simulink model "Main_SpeedOptimisedVersionTannenweg"  (R2024b)
settings: Solver=ode15s  StartTime=0.0  StopTime=3600*2  FixedStep=0.1  RelTol=0.001
model workspace (MAT data in the model file):
  Ti = 5
  fa = 0.00071
  fd = 0.03
  ips = 36
  ma = 0.0013
  md = 0.04
  roomarea1 = 20
  s = 15
libraries: fl_lib x1434, nesl_utility x105, SimscapeFluids_lib x35
(part 19 of 22)

== system Main_SpeedOptimisedVersionTannenweg/OG1/Raum3/X-Atm ==
  Air-Wall Convection : fl_lib/Thermal/Thermal Elements/Convective Heat Transfer  thermal_type=foundation.enum.constant_variable.constant  area=8.7 m^2  heat_tr_coeff=.8 W/m^2/K  min_heat_tr_coeff=1e-3 W/(K*m^2)  T_specify=off  T_priority=High  T=0 K  T_nominal_specify=off  T_nominal_value=1  T_nominal_unit=K  Q_specify=off  Q_priority=High  Q=0 J/s  Q_nominal_specify=off  Q_nominal_value=1  Q_nominal_unit=W
  Air-Window Convection : fl_lib/Thermal/Thermal Elements/Convective Heat Transfer  thermal_type=foundation.enum.constant_variable.constant  area=3 m^2  heat_tr_coeff=.8 W/m^2/K  min_heat_tr_coeff=1e-3 W/(K*m^2)  T_specify=off  T_priority=High  T=0 K  T_nominal_specify=off  T_nominal_value=1  T_nominal_unit=K  Q_specify=off  Q_priority=High  Q=0 J/s  Q_nominal_specify=off  Q_nominal_value=1  Q_nominal_unit=W
  Atm-Wall Convection : fl_lib/Thermal/Thermal Elements/Convective Heat Transfer  thermal_type=foundation.enum.constant_variable.constant  area=8.7 m^2  heat_tr_coeff=25 W/m^2/K  min_heat_tr_coeff=1e-3 W/(K*m^2)  T_specify=off  T_priority=High  T=0 K  T_nominal_specify=off  T_nominal_value=1  T_nominal_unit=K  Q_specify=off  Q_priority=High  Q=0 J/s  Q_nominal_specify=off  Q_nominal_value=1  Q_nominal_unit=W
  Atm-Window Convection : fl_lib/Thermal/Thermal Elements/Convective Heat Transfer  thermal_type=foundation.enum.constant_variable.constant  area=3 m^2  heat_tr_coeff=25 W/m^2/K  min_heat_tr_coeff=1e-3 W/(K*m^2)  T_specify=off  T_priority=High  T=0 K  T_nominal_specify=off  T_nominal_value=1  T_nominal_unit=K  Q_specify=off  Q_priority=High  Q=0 J/s  Q_nominal_specify=off  Q_nominal_value=1  Q_nominal_unit=W
  Half Wall-Air Conduction : fl_lib/Thermal/Thermal Elements/Conductive Heat Transfer  thermal_type=foundation.enum.ConstantVariableTabulated.Constant  wall_geometry=foundation.enum.ConductionWallGeometry.Planar  area=8.7 m^2  thickness=.16 m  d_in=0.05 m  d_out=0.1 m  L=1 m  th_cond_min=10 W/(K*m)  th_cond=.069 W/m/K  th_cond_TLU=[413, 401, 392, 383, 371, 357, 342] W/(K*m)  temp_TLU=[200, 273, 400, 600, 800, 1000, 1200] K  T_specify=off  T_priority=High  T=0 K  T_nominal_specify=off  T_nominal_value=1  T_nominal_unit=K  Q_specify=off  Q_priority=High  Q=0 J/s  Q_nominal_specify=off  Q_nominal_value=1  Q_nominal_unit=W
  Half Wall-Atm Conduction : fl_lib/Thermal/Thermal Elements/Conductive Heat Transfer  thermal_type=foundation.enum.ConstantVariableTabulated.Constant  wall_geometry=foundation.enum.ConductionWallGeometry.Planar  area=8.7 m^2  thickness=.16 m  d_in=0.05 m  d_out=0.1 m  L=1 m  th_cond_min=10 W/(K*m)  th_cond=.069 W/m/K  th_cond_TLU=[413, 401, 392, 383, 371, 357, 342] W/(K*m)  temp_TLU=[200, 273, 400, 600, 800, 1000, 1200] K  T_specify=off  T_priority=High  T=0 K  T_nominal_specify=off  T_nominal_value=1  T_nominal_unit=K  Q_specify=off  Q_priority=High  Q=0 J/s  Q_nominal_specify=off  Q_nominal_value=1  Q_nominal_unit=W
  Half Window-Air Conduction : fl_lib/Thermal/Thermal Elements/Conductive Heat Transfer  thermal_type=foundation.enum.ConstantVariableTabulated.Constant  wall_geometry=foundation.enum.ConductionWallGeometry.Planar  area=3 m^2  thickness=.027 m  d_in=0.05 m  d_out=0.1 m  L=1 m  th_cond_min=10 W/(K*m)  th_cond=.43 W/m/K  th_cond_TLU=[413, 401, 392, 383, 371, 357, 342] W/(K*m)  temp_TLU=[200, 273, 400, 600, 800, 1000, 1200] K  T_specify=off  T_priority=High  T=0 K  T_nominal_specify=off  T_nominal_value=1  T_nominal_unit=K  Q_specify=off  Q_priority=High  Q=0 J/s  Q_nominal_specify=off  Q_nominal_value=1  Q_nominal_unit=W
  Half Window-Atm Conduction : fl_lib/Thermal/Thermal Elements/Conductive Heat Transfer  thermal_type=foundation.enum.ConstantVariableTabulated.Constant  wall_geometry=foundation.enum.ConductionWallGeometry.Planar  area=3 m^2  thickness=.027 m  d_in=0.05 m  d_out=0.1 m  L=1 m  th_cond_min=10 W/(K*m)  th_cond=.43 W/m/K  th_cond_TLU=[413, 401, 392, 383, 371, 357, 342] W/(K*m)  temp_TLU=[200, 273, 400, 600, 800, 1000, 1200] K  T_specify=off  T_priority=High  T=0 K  T_nominal_specify=off  T_nominal_value=1  T_nominal_unit=K  Q_specify=off  Q_priority=High  Q=0 J/s  Q_nominal_specify=off  Q_nominal_value=1  Q_nominal_unit=W
  Thermal Mass Wall : fl_lib/Thermal/Thermal Elements/Thermal Mass  mass_type=foundation.enum.constant_variable.constant  mass=1500 kg  sp_heat=876 J/kg/K  mass_min=1e-6 kg  num_ports=foundation.enum.numPorts2.one  m_specify=off  m_priority=High  m=1 kg  m_nominal_specify=off  m_nominal_value=1  m_nominal_unit=kg  T_specify=on  T_priority=High  T=Ti degC  T_nominal_specify=off  T_nominal_value=1  T_nominal_unit=K  Q_specify=off  Q_priority=None  Q=0 W  Q_nominal_specify=off  Q_nominal_value=1  Q_nominal_unit=W
  Thermal Mass Window : fl_lib/Thermal/Thermal Elements/Thermal Mass  mass_type=foundation.enum.constant_variable.constant  mass=176 kg  sp_heat=884 J/kg/K  mass_min=1e-6 kg  num_ports=foundation.enum.numPorts2.one  m_specify=off  m_priority=High  m=1 kg  m_nominal_specify=off  m_nominal_value=1  m_nominal_unit=kg  T_specify=on  T_priority=High  T=Ti degC  T_nominal_specify=off  T_nominal_value=1  T_nominal_unit=K  Q_specify=off  Q_priority=None  Q=0 W  Q_nominal_specify=off  Q_nominal_value=1  Q_nominal_unit=W
  Conn1 : PMIOPort  Side=Left
  Conn2 : PMIOPort  Port=2  Side=Right
  connections:
  Air-Wall Convection/RConn1 -- Half Wall-Air Conduction/LConn1
  Air-Window Convection/RConn1 -- Half Window-Air Conduction/LConn1
  Half Wall-Atm Conduction/RConn1 -- Atm-Wall Convection/LConn1
  Half Window-Atm Conduction/RConn1 -- Atm-Window Convection/LConn1
  Atm-Wall Convection/RConn1 -- Conn2/RConn1 -- Atm-Window Convection/RConn1
  Half Wall-Atm Conduction/LConn1 -- Half Wall-Air Conduction/RConn1 -- Thermal Mass Wall/LConn1
  Half Window-Atm Conduction/LConn1 -- Half Window-Air Conduction/RConn1 -- Thermal Mass Window/LConn1
  Conn1/RConn1 -- Air-Wall Convection/LConn1 -- Air-Window Convection/LConn1

== system Main_SpeedOptimisedVersionTannenweg/OG1/Raum4/Heater ==
  valve command : Inport
  Gate Valve (TL)1 : SimscapeFluids_lib/Thermal Liquid/Valves & Orifices/Flow Control Valves/Gate Valve (TL)  diam_orifice=fd m  S_min=0 m  area_leak=1e-10 m^2  smoothing_factor=0.01  area=fa m^2  Cd=0.64  Re_c=150
      settings: InternalSimscapePortConfiguration="{\"Bottom\":[],\"Left\":[{\"id\":\"A\",\"label\":\"A\",\"type\":\"foundation.thermal_liquid.thermal_liquid\"},{\"id\":\"S\",\"label\":\"S\",\"type\":\"input\"}],\"Right\":[{\"id\":\"B\",\"label\":\"B\",\"type\":\"foundation.thermal_liquid.thermal_liquid\"}],\"Top\":[]}"
  Subsystem : Subsystem
  heating panel typ 11 : fl_lib/Thermal Liquid/Elements/Pipe (TL)  length=5 m  area=0.01 m^2  Dh=0.1128 m  length_add=1 m  roughness=15e-6 m  Re_lam=2000  Re_tur=4000  shape_factor=64  Nu_lam=3.66  dynamic_compressibility=true  inertia=false  p0=0.101325 MPa  T0=293.15 K  mdot0=0 kg/s
  Water in : PMIOPort  Side=Left
  Heat : PMIOPort  Port=2  Side=Right
  water out : PMIOPort  Port=3  Side=Right
  wires:
  valve command/1 -> Subsystem/1(VCmd)
  connections:
  heating panel typ 11/RConn1 -- water out/RConn1
  Gate Valve (TL)1/RConn1 -- heating panel typ 11/LConn1
  heating panel typ 11/LConn2 -- Heat/RConn1
  Gate Valve (TL)1/LConn2 -- Subsystem/RConn1
  Water in/RConn1 -- Gate Valve (TL)1/LConn1

== system Main_SpeedOptimisedVersionTannenweg/OG1/Raum4/Temp. Sensor ==
  PS2S : nesl_utility/PS-Simulink Converter  PhysicalDomain=network_engine_domain  SubClassName=ps_output  LeftPortType=input  RightPortType=output  PseudoPeriodic=off  Frequencies=[]  VectorFormat=1-D array  Unit=degC  AffineConversion=on
  TRef : fl_lib/Thermal/Thermal Elements/Thermal Reference
  Temperature Sensor : fl_lib/Thermal/Thermal Sensors/Temperature Sensor  temperature_measure=foundation.enum.MeasurementReference.difference
  Pr : PMIOPort  Side=Left
  T : Outport  VectorParamsAs1DForOutWhenUnconnected=off
  wires:
  PS2S/1 -> T/1
  connections:
  Temperature Sensor/RConn1 -- TRef/LConn1
  PS2S/LConn1 -- Temperature Sensor/RConn2
  Pr/RConn1 -- Temperature Sensor/LConn1

== system Main_SpeedOptimisedVersionTannenweg/OG1/Raum4/X-Atm ==
  Air-Wall Convection : fl_lib/Thermal/Thermal Elements/Convective Heat Transfer  thermal_type=foundation.enum.constant_variable.constant  area=4 m^2  heat_tr_coeff=.8 W/m^2/K  min_heat_tr_coeff=1e-3 W/(K*m^2)  T_specify=off  T_priority=High  T=0 K  T_nominal_specify=off  T_nominal_value=1  T_nominal_unit=K  Q_specify=off  Q_priority=High  Q=0 J/s  Q_nominal_specify=off  Q_nominal_value=1  Q_nominal_unit=W
  Air-Window Convection : fl_lib/Thermal/Thermal Elements/Convective Heat Transfer  thermal_type=foundation.enum.constant_variable.constant  area=1.3 m^2  heat_tr_coeff=.8 W/m^2/K  min_heat_tr_coeff=1e-3 W/(K*m^2)  T_specify=off  T_priority=High  T=0 K  T_nominal_specify=off  T_nominal_value=1  T_nominal_unit=K  Q_specify=off  Q_priority=High  Q=0 J/s  Q_nominal_specify=off  Q_nominal_value=1  Q_nominal_unit=W
  Atm-Wall Convection : fl_lib/Thermal/Thermal Elements/Convective Heat Transfer  thermal_type=foundation.enum.constant_variable.constant  area=4 m^2  heat_tr_coeff=25 W/m^2/K  min_heat_tr_coeff=1e-3 W/(K*m^2)  T_specify=off  T_priority=High  T=0 K  T_nominal_specify=off  T_nominal_value=1  T_nominal_unit=K  Q_specify=off  Q_priority=High  Q=0 J/s  Q_nominal_specify=off  Q_nominal_value=1  Q_nominal_unit=W
  Atm-Window Convection : fl_lib/Thermal/Thermal Elements/Convective Heat Transfer  thermal_type=foundation.enum.constant_variable.constant  area=1.3 m^2  heat_tr_coeff=25 W/m^2/K  min_heat_tr_coeff=1e-3 W/(K*m^2)  T_specify=off  T_priority=High  T=0 K  T_nominal_specify=off  T_nominal_value=1  T_nominal_unit=K  Q_specify=off  Q_priority=High  Q=0 J/s  Q_nominal_specify=off  Q_nominal_value=1  Q_nominal_unit=W
  Half Wall-Air Conduction : fl_lib/Thermal/Thermal Elements/Conductive Heat Transfer  thermal_type=foundation.enum.ConstantVariableTabulated.Constant  wall_geometry=foundation.enum.ConductionWallGeometry.Planar  area=4 m^2  thickness=.16 m  d_in=0.05 m  d_out=0.1 m  L=1 m  th_cond_min=10 W/(K*m)  th_cond=.069 W/m/K  th_cond_TLU=[413, 401, 392, 383, 371, 357, 342] W/(K*m)  temp_TLU=[200, 273, 400, 600, 800, 1000, 1200] K  T_specify=off  T_priority=High  T=0 K  T_nominal_specify=off  T_nominal_value=1  T_nominal_unit=K  Q_specify=off  Q_priority=High  Q=0 J/s  Q_nominal_specify=off  Q_nominal_value=1  Q_nominal_unit=W
  Half Wall-Atm Conduction : fl_lib/Thermal/Thermal Elements/Conductive Heat Transfer  thermal_type=foundation.enum.ConstantVariableTabulated.Constant  wall_geometry=foundation.enum.ConductionWallGeometry.Planar  area=4 m^2  thickness=.16 m  d_in=0.05 m  d_out=0.1 m  L=1 m  th_cond_min=10 W/(K*m)  th_cond=.069 W/m/K  th_cond_TLU=[413, 401, 392, 383, 371, 357, 342] W/(K*m)  temp_TLU=[200, 273, 400, 600, 800, 1000, 1200] K  T_specify=off  T_priority=High  T=0 K  T_nominal_specify=off  T_nominal_value=1  T_nominal_unit=K  Q_specify=off  Q_priority=High  Q=0 J/s  Q_nominal_specify=off  Q_nominal_value=1  Q_nominal_unit=W
  Half Window-Air Conduction : fl_lib/Thermal/Thermal Elements/Conductive Heat Transfer  thermal_type=foundation.enum.ConstantVariableTabulated.Constant  wall_geometry=foundation.enum.ConductionWallGeometry.Planar  area=1.3 m^2  thickness=.027 m  d_in=0.05 m  d_out=0.1 m  L=1 m  th_cond_min=10 W/(K*m)  th_cond=.43 W/m/K  th_cond_TLU=[413, 401, 392, 383, 371, 357, 342] W/(K*m)  temp_TLU=[200, 273, 400, 600, 800, 1000, 1200] K  T_specify=off  T_priority=High  T=0 K  T_nominal_specify=off  T_nominal_value=1  T_nominal_unit=K  Q_specify=off  Q_priority=High  Q=0 J/s  Q_nominal_specify=off  Q_nominal_value=1  Q_nominal_unit=W
  Half Window-Atm Conduction : fl_lib/Thermal/Thermal Elements/Conductive Heat Transfer  thermal_type=foundation.enum.ConstantVariableTabulated.Constant  wall_geometry=foundation.enum.ConductionWallGeometry.Planar  area=1.3 m^2  thickness=.027 m  d_in=0.05 m  d_out=0.1 m  L=1 m  th_cond_min=10 W/(K*m)  th_cond=.43 W/m/K  th_cond_TLU=[413, 401, 392, 383, 371, 357, 342] W/(K*m)  temp_TLU=[200, 273, 400, 600, 800, 1000, 1200] K  T_specify=off  T_priority=High  T=0 K  T_nominal_specify=off  T_nominal_value=1  T_nominal_unit=K  Q_specify=off  Q_priority=High  Q=0 J/s  Q_nominal_specify=off  Q_nominal_value=1  Q_nominal_unit=W
  Thermal Mass Wall : fl_lib/Thermal/Thermal Elements/Thermal Mass  mass_type=foundation.enum.constant_variable.constant  mass=706 kg  sp_heat=876 J/kg/K  mass_min=1e-6 kg  num_ports=foundation.enum.numPorts2.one  m_specify=off  m_priority=High  m=1 kg  m_nominal_specify=off  m_nominal_value=1  m_nominal_unit=kg  T_specify=on  T_priority=High  T=Ti degC  T_nominal_specify=off  T_nominal_value=1  T_nominal_unit=K  Q_specify=off  Q_priority=None  Q=0 W  Q_nominal_specify=off  Q_nominal_value=1  Q_nominal_unit=W
  Thermal Mass Window1 : fl_lib/Thermal/Thermal Elements/Thermal Mass  mass_type=foundation.enum.constant_variable.constant  mass=74 kg  sp_heat=884 J/kg/K  mass_min=1e-6 kg  num_ports=foundation.enum.numPorts2.one  m_specify=off  m_priority=High  m=1 kg  m_nominal_specify=off  m_nominal_value=1  m_nominal_unit=kg  T_specify=on  T_priority=High  T=Ti degC  T_nominal_specify=off  T_nominal_value=1  T_nominal_unit=K  Q_specify=off  Q_priority=None  Q=0 W  Q_nominal_specify=off  Q_nominal_value=1  Q_nominal_unit=W
  Conn1 : PMIOPort  Side=Left
  Conn2 : PMIOPort  Port=2  Side=Right
  connections:
  Air-Window Convection/RConn1 -- Half Window-Air Conduction/LConn1
  Air-Wall Convection/RConn1 -- Half Wall-Air Conduction/LConn1
  Half Window-Atm Conduction/RConn1 -- Atm-Window Convection/LConn1
  Half Wall-Atm Conduction/RConn1 -- Atm-Wall Convection/LConn1
  Half Window-Atm Conduction/LConn1 -- Thermal Mass Window1/LConn1 -- Half Window-Air Conduction/RConn1
  Half Wall-Atm Conduction/LConn1 -- Thermal Mass Wall/LConn1 -- Half Wall-Air Conduction/RConn1
  Conn1/RConn1 -- Air-Window Convection/LConn1 -- Air-Wall Convection/LConn1
  Atm-Wall Convection/RConn1 -- Atm-Window Convection/RConn1 -- Conn2/RConn1

== system Main_SpeedOptimisedVersionTannenweg/OG1/Raum5/Heater ==
  valve command : Inport
  Gate Valve (TL)1 : SimscapeFluids_lib/Thermal Liquid/Valves & Orifices/Flow Control Valves/Gate Valve (TL)  diam_orifice=fd m  S_min=0 m  area_leak=1e-10 m^2  smoothing_factor=0.01  area=fa m^2  Cd=0.64  Re_c=150
      settings: InternalSimscapePortConfiguration="{\"Bottom\":[],\"Left\":[{\"id\":\"A\",\"label\":\"A\",\"type\":\"foundation.thermal_liquid.thermal_liquid\"},{\"id\":\"S\",\"label\":\"S\",\"type\":\"input\"}],\"Right\":[{\"id\":\"B\",\"label\":\"B\",\"type\":\"foundation.thermal_liquid.thermal_liquid\"}],\"Top\":[]}"
  Subsystem : Subsystem
  heating panel typ 11 : fl_lib/Thermal Liquid/Elements/Pipe (TL)  length=5 m  area=0.01 m^2  Dh=0.1128 m  length_add=1 m  roughness=15e-6 m  Re_lam=2000  Re_tur=4000  shape_factor=64  Nu_lam=3.66  dynamic_compressibility=true  inertia=false  p0=0.101325 MPa  T0=293.15 K  mdot0=0 kg/s
  Water in : PMIOPort  Side=Left
  Heat : PMIOPort  Port=2  Side=Right
  water out : PMIOPort  Port=3  Side=Right
  wires:
  valve command/1 -> Subsystem/1(VCmd)
  connections:
  heating panel typ 11/LConn2 -- Heat/RConn1
  Gate Valve (TL)1/RConn1 -- heating panel typ 11/LConn1
  heating panel typ 11/RConn1 -- water out/RConn1
  Gate Valve (TL)1/LConn2 -- Subsystem/RConn1
  Water in/RConn1 -- Gate Valve (TL)1/LConn1

== system Main_SpeedOptimisedVersionTannenweg/OG1/Raum5/Temp. Sensor ==
  PS2S : nesl_utility/PS-Simulink Converter  PhysicalDomain=network_engine_domain  SubClassName=ps_output  LeftPortType=input  RightPortType=output  PseudoPeriodic=off  Frequencies=[]  VectorFormat=1-D array  Unit=degC  AffineConversion=on
  TRef : fl_lib/Thermal/Thermal Elements/Thermal Reference
  Temperature Sensor : fl_lib/Thermal/Thermal Sensors/Temperature Sensor  temperature_measure=foundation.enum.MeasurementReference.difference
  Pr : PMIOPort  Side=Left
  T : Outport  VectorParamsAs1DForOutWhenUnconnected=off
  wires:
  PS2S/1 -> T/1
  connections:
  Pr/RConn1 -- Temperature Sensor/LConn1
  PS2S/LConn1 -- Temperature Sensor/RConn2
  Temperature Sensor/RConn1 -- TRef/LConn1

== system Main_SpeedOptimisedVersionTannenweg/OG1/Raum5/X-Atm ==
  Air-Wall Convection : fl_lib/Thermal/Thermal Elements/Convective Heat Transfer  thermal_type=foundation.enum.constant_variable.constant  area=19.2 m^2  heat_tr_coeff=.8 W/m^2/K  min_heat_tr_coeff=1e-3 W/(K*m^2)  T_specify=off  T_priority=High  T=0 K  T_nominal_specify=off  T_nominal_value=1  T_nominal_unit=K  Q_specify=off  Q_priority=High  Q=0 J/s  Q_nominal_specify=off  Q_nominal_value=1  Q_nominal_unit=W
  Air-Window Convection : fl_lib/Thermal/Thermal Elements/Convective Heat Transfer  thermal_type=foundation.enum.constant_variable.constant  area=3.6 m^2  heat_tr_coeff=.8 W/m^2/K  min_heat_tr_coeff=1e-3 W/(K*m^2)  T_specify=off  T_priority=High  T=0 K  T_nominal_specify=off  T_nominal_value=1  T_nominal_unit=K  Q_specify=off  Q_priority=High  Q=0 J/s  Q_nominal_specify=off  Q_nominal_value=1  Q_nominal_unit=W
  Atm-Wall Convection : fl_lib/Thermal/Thermal Elements/Convective Heat Transfer  thermal_type=foundation.enum.constant_variable.constant  area=19.2 m^2  heat_tr_coeff=25 W/m^2/K  min_heat_tr_coeff=1e-3 W/(K*m^2)  T_specify=off  T_priority=High  T=0 K  T_nominal_specify=off  T_nominal_value=1  T_nominal_unit=K  Q_specify=off  Q_priority=High  Q=0 J/s  Q_nominal_specify=off  Q_nominal_value=1  Q_nominal_unit=W
  Atm-Window Convection : fl_lib/Thermal/Thermal Elements/Convective Heat Transfer  thermal_type=foundation.enum.constant_variable.constant  area=3.6 m^2  heat_tr_coeff=25 W/m^2/K  min_heat_tr_coeff=1e-3 W/(K*m^2)  T_specify=off  T_priority=High  T=0 K  T_nominal_specify=off  T_nominal_value=1  T_nominal_unit=K  Q_specify=off  Q_priority=High  Q=0 J/s  Q_nominal_specify=off  Q_nominal_value=1  Q_nominal_unit=W
  Half Wall-Air Conduction : fl_lib/Thermal/Thermal Elements/Conductive Heat Transfer  thermal_type=foundation.enum.ConstantVariableTabulated.Constant  wall_geometry=foundation.enum.ConductionWallGeometry.Planar  area=19.2 m^2  thickness=.16 m  d_in=0.05 m  d_out=0.1 m  L=1 m  th_cond_min=10 W/(K*m)  th_cond=.069 W/m/K  th_cond_TLU=[413, 401, 392, 383, 371, 357, 342] W/(K*m)  temp_TLU=[200, 273, 400, 600, 800, 1000, 1200] K  T_specify=off  T_priority=High  T=0 K  T_nominal_specify=off  T_nominal_value=1  T_nominal_unit=K  Q_specify=off  Q_priority=High  Q=0 J/s  Q_nominal_specify=off  Q_nominal_value=1  Q_nominal_unit=W
  Half Wall-Atm Conduction : fl_lib/Thermal/Thermal Elements/Conductive Heat Transfer  thermal_type=foundation.enum.ConstantVariableTabulated.Constant  wall_geometry=foundation.enum.ConductionWallGeometry.Planar  area=19.2 m^2  thickness=.16 m  d_in=0.05 m  d_out=0.1 m  L=1 m  th_cond_min=10 W/(K*m)  th_cond=.069 W/m/K  th_cond_TLU=[413, 401, 392, 383, 371, 357, 342] W/(K*m)  temp_TLU=[200, 273, 400, 600, 800, 1000, 1200] K  T_specify=off  T_priority=High  T=0 K  T_nominal_specify=off  T_nominal_value=1  T_nominal_unit=K  Q_specify=off  Q_priority=High  Q=0 J/s  Q_nominal_specify=off  Q_nominal_value=1  Q_nominal_unit=W
  Half Window-Air Conduction : fl_lib/Thermal/Thermal Elements/Conductive Heat Transfer  thermal_type=foundation.enum.ConstantVariableTabulated.Constant  wall_geometry=foundation.enum.ConductionWallGeometry.Planar  area=3.6 m^2  thickness=.027 m  d_in=0.05 m  d_out=0.1 m  L=1 m  th_cond_min=10 W/(K*m)  th_cond=.43 W/m/K  th_cond_TLU=[413, 401, 392, 383, 371, 357, 342] W/(K*m)  temp_TLU=[200, 273, 400, 600, 800, 1000, 1200] K  T_specify=off  T_priority=High  T=0 K  T_nominal_specify=off  T_nominal_value=1  T_nominal_unit=K  Q_specify=off  Q_priority=High  Q=0 J/s  Q_nominal_specify=off  Q_nominal_value=1  Q_nominal_unit=W
  Half Window-Atm Conduction : fl_lib/Thermal/Thermal Elements/Conductive Heat Transfer  thermal_type=foundation.enum.ConstantVariableTabulated.Constant  wall_geometry=foundation.enum.ConductionWallGeometry.Planar  area=3.6 m^2  thickness=.027 m  d_in=0.05 m  d_out=0.1 m  L=1 m  th_cond_min=10 W/(K*m)  th_cond=.43 W/m/K  th_cond_TLU=[413, 401, 392, 383, 371, 357, 342] W/(K*m)  temp_TLU=[200, 273, 400, 600, 800, 1000, 1200] K  T_specify=off  T_priority=High  T=0 K  T_nominal_specify=off  T_nominal_value=1  T_nominal_unit=K  Q_specify=off  Q_priority=High  Q=0 J/s  Q_nominal_specify=off  Q_nominal_value=1  Q_nominal_unit=W
  Thermal Mass Wall : fl_lib/Thermal/Thermal Elements/Thermal Mass  mass_type=foundation.enum.constant_variable.constant  mass=19.2*.3*547 kg  sp_heat=876 J/kg/K  mass_min=1e-6 kg  num_ports=foundation.enum.numPorts2.one  m_specify=off  m_priority=High  m=1 kg  m_nominal_specify=off  m_nominal_value=1  m_nominal_unit=kg  T_specify=on  T_priority=High  T=Ti degC  T_nominal_specify=off  T_nominal_value=1  T_nominal_unit=K  Q_specify=off  Q_priority=None  Q=0 W  Q_nominal_specify=off  Q_nominal_value=1  Q_nominal_unit=W
  Thermal Mass Window : fl_lib/Thermal/Thermal Elements/Thermal Mass  mass_type=foundation.enum.constant_variable.constant  mass=3.6*56.8 kg  sp_heat=884 J/kg/K  mass_min=1e-6 kg  num_ports=foundation.enum.numPorts2.one  m_specify=off  m_priority=High  m=1 kg  m_nominal_specify=off  m_nominal_value=1  m_nominal_unit=kg  T_specify=on  T_priority=High  T=Ti degC  T_nominal_specify=off  T_nominal_value=1  T_nominal_unit=K  Q_specify=off  Q_priority=None  Q=0 W  Q_nominal_specify=off  Q_nominal_value=1  Q_nominal_unit=W
  Conn1 : PMIOPort  Side=Left
  Conn2 : PMIOPort  Port=2  Side=Right
  connections:
  Air-Window Convection/RConn1 -- Half Window-Air Conduction/LConn1
  Half Window-Atm Conduction/RConn1 -- Atm-Window Convection/LConn1
  Half Wall-Atm Conduction/RConn1 -- Atm-Wall Convection/LConn1
  Air-Wall Convection/RConn1 -- Half Wall-Air Conduction/LConn1
  Half Wall-Atm Conduction/LConn1 -- Thermal Mass Wall/LConn1 -- Half Wall-Air Conduction/RConn1
  Half Window-Atm Conduction/LConn1 -- Thermal Mass Window/LConn1 -- Half Window-Air Conduction/RConn1
  Conn2/RConn1 -- Atm-Wall Convection/RConn1 -- Atm-Window Convection/RConn1
  Conn1/RConn1 -- Air-Wall Convection/LConn1 -- Air-Window Convection/LConn1

== system Main_SpeedOptimisedVersionTannenweg/OG1/Raum6/Heater ==
  valve command : Inport
  Gate Valve (TL)1 : SimscapeFluids_lib/Thermal Liquid/Valves & Orifices/Flow Control Valves/Gate Valve (TL)  diam_orifice=fd m  S_min=0 m  area_leak=1e-10 m^2  smoothing_factor=0.01  area=fa m^2  Cd=0.64  Re_c=150
      settings: InternalSimscapePortConfiguration="{\"Bottom\":[],\"Left\":[{\"id\":\"A\",\"label\":\"A\",\"type\":\"foundation.thermal_liquid.thermal_liquid\"},{\"id\":\"S\",\"label\":\"S\",\"type\":\"input\"}],\"Right\":[{\"id\":\"B\",\"label\":\"B\",\"type\":\"foundation.thermal_liquid.thermal_liquid\"}],\"Top\":[]}"
  Subsystem : Subsystem
  heating panel typ 11 : fl_lib/Thermal Liquid/Elements/Pipe (TL)  length=5 m  area=0.01 m^2  Dh=0.1128 m  length_add=1 m  roughness=15e-6 m  Re_lam=2000  Re_tur=4000  shape_factor=64  Nu_lam=3.66  dynamic_compressibility=true  inertia=false  p0=0.101325 MPa  T0=293.15 K  mdot0=0 kg/s
  Water in : PMIOPort  Side=Left
  Heat : PMIOPort  Port=2  Side=Right
  water out : PMIOPort  Port=3  Side=Right
  wires:
  valve command/1 -> Subsystem/1(VCmd)
  connections:
  heating panel typ 11/RConn1 -- water out/RConn1
  Gate Valve (TL)1/RConn1 -- heating panel typ 11/LConn1
  heating panel typ 11/LConn2 -- Heat/RConn1
  Gate Valve (TL)1/LConn2 -- Subsystem/RConn1
  Water in/RConn1 -- Gate Valve (TL)1/LConn1

== system Main_SpeedOptimisedVersionTannenweg/OG1/Raum6/Temp. Sensor ==
  PS2S : nesl_utility/PS-Simulink Converter  PhysicalDomain=network_engine_domain  SubClassName=ps_output  LeftPortType=input  RightPortType=output  PseudoPeriodic=off  Frequencies=[]  VectorFormat=1-D array  Unit=degC  AffineConversion=on
  TRef : fl_lib/Thermal/Thermal Elements/Thermal Reference
  Temperature Sensor : fl_lib/Thermal/Thermal Sensors/Temperature Sensor  temperature_measure=foundation.enum.MeasurementReference.difference
  Pr : PMIOPort  Side=Left
  T : Outport  VectorParamsAs1DForOutWhenUnconnected=off
  wires:
  PS2S/1 -> T/1
  connections:
  Temperature Sensor/RConn1 -- TRef/LConn1
  PS2S/LConn1 -- Temperature Sensor/RConn2
  Pr/RConn1 -- Temperature Sensor/LConn1

== system Main_SpeedOptimisedVersionTannenweg/OG1/Raum6/X-Atm ==
  Air-Wall Convection : fl_lib/Thermal/Thermal Elements/Convective Heat Transfer  thermal_type=foundation.enum.constant_variable.constant  area=5.6 m^2  heat_tr_coeff=.8 W/m^2/K  min_heat_tr_coeff=1e-3 W/(K*m^2)  T_specify=off  T_priority=High  T=0 K  T_nominal_specify=off  T_nominal_value=1  T_nominal_unit=K  Q_specify=off  Q_priority=High  Q=0 J/s  Q_nominal_specify=off  Q_nominal_value=1  Q_nominal_unit=W
  Air-Window Convection : fl_lib/Thermal/Thermal Elements/Convective Heat Transfer  thermal_type=foundation.enum.constant_variable.constant  area=1.3 m^2  heat_tr_coeff=.8 W/m^2/K  min_heat_tr_coeff=1e-3 W/(K*m^2)  T_specify=off  T_priority=High  T=0 K  T_nominal_specify=off  T_nominal_value=1  T_nominal_unit=K  Q_specify=off  Q_priority=High  Q=0 J/s  Q_nominal_specify=off  Q_nominal_value=1  Q_nominal_unit=W
  Atm-Wall Convection : fl_lib/Thermal/Thermal Elements/Convective Heat Transfer  thermal_type=foundation.enum.constant_variable.constant  area=5.6 m^2  heat_tr_coeff=25 W/m^2/K  min_heat_tr_coeff=1e-3 W/(K*m^2)  T_specify=off  T_priority=High  T=0 K  T_nominal_specify=off  T_nominal_value=1  T_nominal_unit=K  Q_specify=off  Q_priority=High  Q=0 J/s  Q_nominal_specify=off  Q_nominal_value=1  Q_nominal_unit=W
  Atm-Window Convection : fl_lib/Thermal/Thermal Elements/Convective Heat Transfer  thermal_type=foundation.enum.constant_variable.constant  area=1.3 m^2  heat_tr_coeff=25 W/m^2/K  min_heat_tr_coeff=1e-3 W/(K*m^2)  T_specify=off  T_priority=High  T=0 K  T_nominal_specify=off  T_nominal_value=1  T_nominal_unit=K  Q_specify=off  Q_priority=High  Q=0 J/s  Q_nominal_specify=off  Q_nominal_value=1  Q_nominal_unit=W
  Half Wall-Air Conduction : fl_lib/Thermal/Thermal Elements/Conductive Heat Transfer  thermal_type=foundation.enum.ConstantVariableTabulated.Constant  wall_geometry=foundation.enum.ConductionWallGeometry.Planar  area=5.6 m^2  thickness=.16 m  d_in=0.05 m  d_out=0.1 m  L=1 m  th_cond_min=10 W/(K*m)  th_cond=.069 W/m/K  th_cond_TLU=[413, 401, 392, 383, 371, 357, 342] W/(K*m)  temp_TLU=[200, 273, 400, 600, 800, 1000, 1200] K  T_specify=off  T_priority=High  T=0 K  T_nominal_specify=off  T_nominal_value=1  T_nominal_unit=K  Q_specify=off  Q_priority=High  Q=0 J/s  Q_nominal_specify=off  Q_nominal_value=1  Q_nominal_unit=W
  Half Wall-Atm Conduction : fl_lib/Thermal/Thermal Elements/Conductive Heat Transfer  thermal_type=foundation.enum.ConstantVariableTabulated.Constant  wall_geometry=foundation.enum.ConductionWallGeometry.Planar  area=5.6 m^2  thickness=.16 m  d_in=0.05 m  d_out=0.1 m  L=1 m  th_cond_min=10 W/(K*m)  th_cond=.069 W/m/K  th_cond_TLU=[413, 401, 392, 383, 371, 357, 342] W/(K*m)  temp_TLU=[200, 273, 400, 600, 800, 1000, 1200] K  T_specify=off  T_priority=High  T=0 K  T_nominal_specify=off  T_nominal_value=1  T_nominal_unit=K  Q_specify=off  Q_priority=High  Q=0 J/s  Q_nominal_specify=off  Q_nominal_value=1  Q_nominal_unit=W
  Half Window-Air Conduction : fl_lib/Thermal/Thermal Elements/Conductive Heat Transfer  thermal_type=foundation.enum.ConstantVariableTabulated.Constant  wall_geometry=foundation.enum.ConductionWallGeometry.Planar  area=1.3 m^2  thickness=.027 m  d_in=0.05 m  d_out=0.1 m  L=1 m  th_cond_min=10 W/(K*m)  th_cond=.43 W/m/K  th_cond_TLU=[413, 401, 392, 383, 371, 357, 342] W/(K*m)  temp_TLU=[200, 273, 400, 600, 800, 1000, 1200] K  T_specify=off  T_priority=High  T=0 K  T_nominal_specify=off  T_nominal_value=1  T_nominal_unit=K  Q_specify=off  Q_priority=High  Q=0 J/s  Q_nominal_specify=off  Q_nominal_value=1  Q_nominal_unit=W
  Half Window-Atm Conduction : fl_lib/Thermal/Thermal Elements/Conductive Heat Transfer  thermal_type=foundation.enum.ConstantVariableTabulated.Constant  wall_geometry=foundation.enum.ConductionWallGeometry.Planar  area=1.3 m^2  thickness=.027 m  d_in=0.05 m  d_out=0.1 m  L=1 m  th_cond_min=10 W/(K*m)  th_cond=.43 W/m/K  th_cond_TLU=[413, 401, 392, 383, 371, 357, 342] W/(K*m)  temp_TLU=[200, 273, 400, 600, 800, 1000, 1200] K  T_specify=off  T_priority=High  T=0 K  T_nominal_specify=off  T_nominal_value=1  T_nominal_unit=K  Q_specify=off  Q_priority=High  Q=0 J/s  Q_nominal_specify=off  Q_nominal_value=1  Q_nominal_unit=W
  Thermal Mass Wall : fl_lib/Thermal/Thermal Elements/Thermal Mass  mass_type=foundation.enum.constant_variable.constant  mass=5.6*164 kg  sp_heat=876 J/kg/K  mass_min=1e-6 kg  num_ports=foundation.enum.numPorts2.one  m_specify=off  m_priority=High  m=1 kg  m_nominal_specify=off  m_nominal_value=1  m_nominal_unit=kg  T_specify=on  T_priority=High  T=Ti degC  T_nominal_specify=off  T_nominal_value=1  T_nominal_unit=K  Q_specify=off  Q_priority=None  Q=0 W  Q_nominal_specify=off  Q_nominal_value=1  Q_nominal_unit=W
  Thermal Mass Window : fl_lib/Thermal/Thermal Elements/Thermal Mass  mass_type=foundation.enum.constant_variable.constant  mass=1.3*56.8 kg  sp_heat=884 J/kg/K  mass_min=1e-6 kg  num_ports=foundation.enum.numPorts2.one  m_specify=off  m_priority=High  m=1 kg  m_nominal_specify=off  m_nominal_value=1  m_nominal_unit=kg  T_specify=on  T_priority=High  T=Ti degC  T_nominal_specify=off  T_nominal_value=1  T_nominal_unit=K  Q_specify=off  Q_priority=None  Q=0 W  Q_nominal_specify=off  Q_nominal_value=1  Q_nominal_unit=W
  Conn1 : PMIOPort  Side=Left
  Conn2 : PMIOPort  Port=2  Side=Right
  connections:
  Air-Wall Convection/RConn1 -- Half Wall-Air Conduction/LConn1
  Air-Window Convection/RConn1 -- Half Window-Air Conduction/LConn1
  Half Wall-Atm Conduction/RConn1 -- Atm-Wall Convection/LConn1
  Half Window-Atm Conduction/RConn1 -- Atm-Window Convection/LConn1
  Half Wall-Atm Conduction/LConn1 -- Thermal Mass Wall/LConn1 -- Half Wall-Air Conduction/RConn1
  Half Window-Atm Conduction/LConn1 -- Thermal Mass Window/LConn1 -- Half Window-Air Conduction/RConn1
  Air-Window Convection/LConn1 -- Air-Wall Convection/LConn1 -- Conn1/RConn1
  Atm-Window Convection/RConn1 -- Atm-Wall Convection/RConn1 -- Conn2/RConn1

== system Main_SpeedOptimisedVersionTannenweg/OG1/Raum7/Heater ==
  valve command : Inport
  Gate Valve (TL)1 : SimscapeFluids_lib/Thermal Liquid/Valves & Orifices/Flow Control Valves/Gate Valve (TL)  diam_orifice=fd m  S_min=0 m  area_leak=1e-10 m^2  smoothing_factor=0.01  area=fa m^2  Cd=0.64  Re_c=150
      settings: InternalSimscapePortConfiguration="{\"Bottom\":[],\"Left\":[{\"id\":\"A\",\"label\":\"A\",\"type\":\"foundation.thermal_liquid.thermal_liquid\"},{\"id\":\"S\",\"label\":\"S\",\"type\":\"input\"}],\"Right\":[{\"id\":\"B\",\"label\":\"B\",\"type\":\"foundation.thermal_liquid.thermal_liquid\"}],\"Top\":[]}"
  Subsystem : Subsystem
  heating panel typ 11 : fl_lib/Thermal Liquid/Elements/Pipe (TL)  length=5 m  area=0.01 m^2  Dh=0.1128 m  length_add=1 m  roughness=15e-6 m  Re_lam=2000  Re_tur=4000  shape_factor=64  Nu_lam=3.66  dynamic_compressibility=true  inertia=false  p0=0.101325 MPa  T0=293.15 K  mdot0=0 kg/s
  Water in : PMIOPort  Side=Left
  Heat : PMIOPort  Port=2  Side=Right
  water out : PMIOPort  Port=3  Side=Right
  wires:
  valve command/1 -> Subsystem/1(VCmd)
  connections:
  heating panel typ 11/LConn2 -- Heat/RConn1
  Gate Valve (TL)1/RConn1 -- heating panel typ 11/LConn1
  heating panel typ 11/RConn1 -- water out/RConn1
  Subsystem/RConn1 -- Gate Valve (TL)1/LConn2
  Water in/RConn1 -- Gate Valve (TL)1/LConn1

== system Main_SpeedOptimisedVersionTannenweg/OG1/Raum7/Temp. Sensor ==
  PS2S : nesl_utility/PS-Simulink Converter  PhysicalDomain=network_engine_domain  SubClassName=ps_output  LeftPortType=input  RightPortType=output  PseudoPeriodic=off  Frequencies=[]  VectorFormat=1-D array  Unit=degC  AffineConversion=on
  TRef : fl_lib/Thermal/Thermal Elements/Thermal Reference
  Temperature Sensor : fl_lib/Thermal/Thermal Sensors/Temperature Sensor  temperature_measure=foundation.enum.MeasurementReference.difference
  Pr : PMIOPort  Side=Left
  T : Outport  VectorParamsAs1DForOutWhenUnconnected=off
  wires:
  PS2S/1 -> T/1
  connections:
  Pr/RConn1 -- Temperature Sensor/LConn1
  PS2S/LConn1 -- Temperature Sensor/RConn2
  Temperature Sensor/RConn1 -- TRef/LConn1

== system Main_SpeedOptimisedVersionTannenweg/OG1/Raum8/Heater ==
  valve command : Inport
  Gate Valve (TL)1 : SimscapeFluids_lib/Thermal Liquid/Valves & Orifices/Flow Control Valves/Gate Valve (TL)  diam_orifice=fd m  S_min=0 m  area_leak=1e-10 m^2  smoothing_factor=0.01  area=fa m^2  Cd=0.64  Re_c=150
      settings: InternalSimscapePortConfiguration="{\"Bottom\":[],\"Left\":[{\"id\":\"A\",\"label\":\"A\",\"type\":\"foundation.thermal_liquid.thermal_liquid\"},{\"id\":\"S\",\"label\":\"S\",\"type\":\"input\"}],\"Right\":[{\"id\":\"B\",\"label\":\"B\",\"type\":\"foundation.thermal_liquid.thermal_liquid\"}],\"Top\":[]}"
  Subsystem : Subsystem
  heating panel typ 11 : fl_lib/Thermal Liquid/Elements/Pipe (TL)  length=5 m  area=0.01 m^2  Dh=0.1128 m  length_add=1 m  roughness=15e-6 m  Re_lam=2000  Re_tur=4000  shape_factor=64  Nu_lam=3.66  dynamic_compressibility=true  inertia=false  p0=0.101325 MPa  T0=293.15 K  mdot0=0 kg/s
  Water in : PMIOPort  Side=Left
  Heat : PMIOPort  Port=2  Side=Right
  water out : PMIOPort  Port=3  Side=Right
  wires:
  valve command/1 -> Subsystem/1(VCmd)
  connections:
  heating panel typ 11/LConn2 -- Heat/RConn1
  Gate Valve (TL)1/RConn1 -- heating panel typ 11/LConn1
  heating panel typ 11/RConn1 -- water out/RConn1
  Gate Valve (TL)1/LConn2 -- Subsystem/RConn1
  Water in/RConn1 -- Gate Valve (TL)1/LConn1

== system Main_SpeedOptimisedVersionTannenweg/OG1/Raum8/Temp. Sensor ==
  PS2S : nesl_utility/PS-Simulink Converter  PhysicalDomain=network_engine_domain  SubClassName=ps_output  LeftPortType=input  RightPortType=output  PseudoPeriodic=off  Frequencies=[]  VectorFormat=1-D array  Unit=degC  AffineConversion=on
  TRef : fl_lib/Thermal/Thermal Elements/Thermal Reference
  Temperature Sensor : fl_lib/Thermal/Thermal Sensors/Temperature Sensor  temperature_measure=foundation.enum.MeasurementReference.difference
  Pr : PMIOPort  Side=Left
  T : Outport  VectorParamsAs1DForOutWhenUnconnected=off
  wires:
  PS2S/1 -> T/1
  connections:
  Pr/RConn1 -- Temperature Sensor/LConn1
  PS2S/LConn1 -- Temperature Sensor/RConn2
  Temperature Sensor/RConn1 -- TRef/LConn1

== system Main_SpeedOptimisedVersionTannenweg/OG1/Raum8/X-Atm ==
  Air-Wall Convection : fl_lib/Thermal/Thermal Elements/Convective Heat Transfer  thermal_type=foundation.enum.constant_variable.constant  area=3.7 m^2  heat_tr_coeff=.8 W/m^2/K  min_heat_tr_coeff=1e-3 W/(K*m^2)  T_specify=off  T_priority=High  T=0 K  T_nominal_specify=off  T_nominal_value=1  T_nominal_unit=K  Q_specify=off  Q_priority=High  Q=0 J/s  Q_nominal_specify=off  Q_nominal_value=1  Q_nominal_unit=W
  Air-Window Convection : fl_lib/Thermal/Thermal Elements/Convective Heat Transfer  thermal_type=foundation.enum.constant_variable.constant  area=1.3 m^2  heat_tr_coeff=.8 W/m^2/K  min_heat_tr_coeff=1e-3 W/(K*m^2)  T_specify=off  T_priority=High  T=0 K  T_nominal_specify=off  T_nominal_value=1  T_nominal_unit=K  Q_specify=off  Q_priority=High  Q=0 J/s  Q_nominal_specify=off  Q_nominal_value=1  Q_nominal_unit=W
  Atm-Wall Convection : fl_lib/Thermal/Thermal Elements/Convective Heat Transfer  thermal_type=foundation.enum.constant_variable.constant  area=3.7 m^2  heat_tr_coeff=25 W/m^2/K  min_heat_tr_coeff=1e-3 W/(K*m^2)  T_specify=off  T_priority=High  T=0 K  T_nominal_specify=off  T_nominal_value=1  T_nominal_unit=K  Q_specify=off  Q_priority=High  Q=0 J/s  Q_nominal_specify=off  Q_nominal_value=1  Q_nominal_unit=W
  Atm-Window Convection : fl_lib/Thermal/Thermal Elements/Convective Heat Transfer  thermal_type=foundation.enum.constant_variable.constant  area=1.3 m^2  heat_tr_coeff=25 W/m^2/K  min_heat_tr_coeff=1e-3 W/(K*m^2)  T_specify=off  T_priority=High  T=0 K  T_nominal_specify=off  T_nominal_value=1  T_nominal_unit=K  Q_specify=off  Q_priority=High  Q=0 J/s  Q_nominal_specify=off  Q_nominal_value=1  Q_nominal_unit=W
  Half Wall-Air Conduction : fl_lib/Thermal/Thermal Elements/Conductive Heat Transfer  thermal_type=foundation.enum.ConstantVariableTabulated.Constant  wall_geometry=foundation.enum.ConductionWallGeometry.Planar  area=3.7 m^2  thickness=.16 m  d_in=0.05 m  d_out=0.1 m  L=1 m  th_cond_min=10 W/(K*m)  th_cond=.069 W/m/K  th_cond_TLU=[413, 401, 392, 383, 371, 357, 342] W/(K*m)  temp_TLU=[200, 273, 400, 600, 800, 1000, 1200] K  T_specify=off  T_priority=High  T=0 K  T_nominal_specify=off  T_nominal_value=1  T_nominal_unit=K  Q_specify=off  Q_priority=High  Q=0 J/s  Q_nominal_specify=off  Q_nominal_value=1  Q_nominal_unit=W
  Half Wall-Atm Conduction : fl_lib/Thermal/Thermal Elements/Conductive Heat Transfer  thermal_type=foundation.enum.ConstantVariableTabulated.Constant  wall_geometry=foundation.enum.ConductionWallGeometry.Planar  area=3.7 m^2  thickness=.16 m  d_in=0.05 m  d_out=0.1 m  L=1 m  th_cond_min=10 W/(K*m)  th_cond=.069 W/m/K  th_cond_TLU=[413, 401, 392, 383, 371, 357, 342] W/(K*m)  temp_TLU=[200, 273, 400, 600, 800, 1000, 1200] K  T_specify=off  T_priority=High  T=0 K  T_nominal_specify=off  T_nominal_value=1  T_nominal_unit=K  Q_specify=off  Q_priority=High  Q=0 J/s  Q_nominal_specify=off  Q_nominal_value=1  Q_nominal_unit=W
  Half Window-Air Conduction : fl_lib/Thermal/Thermal Elements/Conductive Heat Transfer  thermal_type=foundation.enum.ConstantVariableTabulated.Constant  wall_geometry=foundation.enum.ConductionWallGeometry.Planar  area=1.3 m^2  thickness=.027 m  d_in=0.05 m  d_out=0.1 m  L=1 m  th_cond_min=10 W/(K*m)  th_cond=.43 W/m/K  th_cond_TLU=[413, 401, 392, 383, 371, 357, 342] W/(K*m)  temp_TLU=[200, 273, 400, 600, 800, 1000, 1200] K  T_specify=off  T_priority=High  T=0 K  T_nominal_specify=off  T_nominal_value=1  T_nominal_unit=K  Q_specify=off  Q_priority=High  Q=0 J/s  Q_nominal_specify=off  Q_nominal_value=1  Q_nominal_unit=W
  Half Window-Atm Conduction : fl_lib/Thermal/Thermal Elements/Conductive Heat Transfer  thermal_type=foundation.enum.ConstantVariableTabulated.Constant  wall_geometry=foundation.enum.ConductionWallGeometry.Planar  area=1.3 m^2  thickness=.027 m  d_in=0.05 m  d_out=0.1 m  L=1 m  th_cond_min=10 W/(K*m)  th_cond=.43 W/m/K  th_cond_TLU=[413, 401, 392, 383, 371, 357, 342] W/(K*m)  temp_TLU=[200, 273, 400, 600, 800, 1000, 1200] K  T_specify=off  T_priority=High  T=0 K  T_nominal_specify=off  T_nominal_value=1  T_nominal_unit=K  Q_specify=off  Q_priority=High  Q=0 J/s  Q_nominal_specify=off  Q_nominal_value=1  Q_nominal_unit=W
  Thermal Mass Wall : fl_lib/Thermal/Thermal Elements/Thermal Mass  mass_type=foundation.enum.constant_variable.constant  mass=3.7*164 kg  sp_heat=876 J/kg/K  mass_min=1e-6 kg  num_ports=foundation.enum.numPorts2.one  m_specify=off  m_priority=High  m=1 kg  m_nominal_specify=off  m_nominal_value=1  m_nominal_unit=kg  T_specify=on  T_priority=High  T=Ti degC  T_nominal_specify=off  T_nominal_value=1  T_nominal_unit=K  Q_specify=off  Q_priority=None  Q=0 W  Q_nominal_specify=off  Q_nominal_value=1  Q_nominal_unit=W
  Thermal Mass Window : fl_lib/Thermal/Thermal Elements/Thermal Mass  mass_type=foundation.enum.constant_variable.constant  mass=1.3*56.8 kg  sp_heat=884 J/kg/K  mass_min=1e-6 kg  num_ports=foundation.enum.numPorts2.one  m_specify=off  m_priority=High  m=1 kg  m_nominal_specify=off  m_nominal_value=1  m_nominal_unit=kg  T_specify=on  T_priority=High  T=Ti degC  T_nominal_specify=off  T_nominal_value=1  T_nominal_unit=K  Q_specify=off  Q_priority=None  Q=0 W  Q_nominal_specify=off  Q_nominal_value=1  Q_nominal_unit=W
  Conn1 : PMIOPort  Side=Left
  Conn2 : PMIOPort  Port=2  Side=Right
  connections:
  Half Window-Atm Conduction/RConn1 -- Atm-Window Convection/LConn1
  Air-Window Convection/RConn1 -- Half Window-Air Conduction/LConn1
  Air-Wall Convection/RConn1 -- Half Wall-Air Conduction/LConn1
  Half Wall-Atm Conduction/RConn1 -- Atm-Wall Convection/LConn1
  Half Wall-Atm Conduction/LConn1 -- Thermal Mass Wall/LConn1 -- Half Wall-Air Conduction/RConn1
  Half Window-Atm Conduction/LConn1 -- Thermal Mass Window/LConn1 -- Half Window-Air Conduction/RConn1
  Atm-Wall Convection/RConn1 -- Conn2/RConn1 -- Atm-Window Convection/RConn1
  Conn1/RConn1 -- Air-Wall Convection/LConn1 -- Air-Window Convection/LConn1

== system Main_SpeedOptimisedVersionTannenweg/OG1/Raum9/Heater ==
  valve command : Inport
  Gate Valve (TL)1 : SimscapeFluids_lib/Thermal Liquid/Valves & Orifices/Flow Control Valves/Gate Valve (TL)  diam_orifice=fd m  S_min=0 m  area_leak=1e-10 m^2  smoothing_factor=0.01  area=fa m^2  Cd=0.64  Re_c=150
      settings: InternalSimscapePortConfiguration="{\"Bottom\":[],\"Left\":[{\"id\":\"A\",\"label\":\"A\",\"type\":\"foundation.thermal_liquid.thermal_liquid\"},{\"id\":\"S\",\"label\":\"S\",\"type\":\"input\"}],\"Right\":[{\"id\":\"B\",\"label\":\"B\",\"type\":\"foundation.thermal_liquid.thermal_liquid\"}],\"Top\":[]}"
  Subsystem : Subsystem
  heating panel typ 11 : fl_lib/Thermal Liquid/Elements/Pipe (TL)  length=5 m  area=0.01 m^2  Dh=0.1128 m  length_add=1 m  roughness=15e-6 m  Re_lam=2000  Re_tur=4000  shape_factor=64  Nu_lam=3.66  dynamic_compressibility=true  inertia=false  p0=0.101325 MPa  T0=293.15 K  mdot0=0 kg/s
  Water in : PMIOPort  Side=Left
  Heat : PMIOPort  Port=2  Side=Right
  water out : PMIOPort  Port=3  Side=Right
  wires:
  valve command/1 -> Subsystem/1(VCmd)
  connections:
  heating panel typ 11/RConn1 -- water out/RConn1
  Gate Valve (TL)1/RConn1 -- heating panel typ 11/LConn1
  heating panel typ 11/LConn2 -- Heat/RConn1
  Gate Valve (TL)1/LConn2 -- Subsystem/RConn1
  Water in/RConn1 -- Gate Valve (TL)1/LConn1

== system Main_SpeedOptimisedVersionTannenweg/OG1/Raum9/Temp. Sensor ==
  PS2S : nesl_utility/PS-Simulink Converter  PhysicalDomain=network_engine_domain  SubClassName=ps_output  LeftPortType=input  RightPortType=output  PseudoPeriodic=off  Frequencies=[]  VectorFormat=1-D array  Unit=degC  AffineConversion=on
  TRef : fl_lib/Thermal/Thermal Elements/Thermal Reference
  Temperature Sensor : fl_lib/Thermal/Thermal Sensors/Temperature Sensor  temperature_measure=foundation.enum.MeasurementReference.difference
  Pr : PMIOPort  Side=Left
  T : Outport  VectorParamsAs1DForOutWhenUnconnected=off
  wires:
  PS2S/1 -> T/1
  connections:
  Temperature Sensor/RConn1 -- TRef/LConn1
  PS2S/LConn1 -- Temperature Sensor/RConn2
  Pr/RConn1 -- Temperature Sensor/LConn1

== system Main_SpeedOptimisedVersionTannenweg/OG1/Raum9/X-Atm ==
  Air-Wall Convection : fl_lib/Thermal/Thermal Elements/Convective Heat Transfer  thermal_type=foundation.enum.constant_variable.constant  area=22 m^2  heat_tr_coeff=.8 W/m^2/K  min_heat_tr_coeff=1e-3 W/(K*m^2)  T_specify=off  T_priority=High  T=0 K  T_nominal_specify=off  T_nominal_value=1  T_nominal_unit=K  Q_specify=off  Q_priority=High  Q=0 J/s  Q_nominal_specify=off  Q_nominal_value=1  Q_nominal_unit=W
  Air-Window Convection : fl_lib/Thermal/Thermal Elements/Convective Heat Transfer  thermal_type=foundation.enum.constant_variable.constant  area=5 m^2  heat_tr_coeff=.8 W/m^2/K  min_heat_tr_coeff=1e-3 W/(K*m^2)  T_specify=off  T_priority=High  T=0 K  T_nominal_specify=off  T_nominal_value=1  T_nominal_unit=K  Q_specify=off  Q_priority=High  Q=0 J/s  Q_nominal_specify=off  Q_nominal_value=1  Q_nominal_unit=W
  Atm-Wall Convection : fl_lib/Thermal/Thermal Elements/Convective Heat Transfer  thermal_type=foundation.enum.constant_variable.constant  area=22 m^2  heat_tr_coeff=25 W/m^2/K  min_heat_tr_coeff=1e-3 W/(K*m^2)  T_specify=off  T_priority=High  T=0 K  T_nominal_specify=off  T_nominal_value=1  T_nominal_unit=K  Q_specify=off  Q_priority=High  Q=0 J/s  Q_nominal_specify=off  Q_nominal_value=1  Q_nominal_unit=W
  Atm-Window Convection : fl_lib/Thermal/Thermal Elements/Convective Heat Transfer  thermal_type=foundation.enum.constant_variable.constant  area=5 m^2  heat_tr_coeff=25 W/m^2/K  min_heat_tr_coeff=1e-3 W/(K*m^2)  T_specify=off  T_priority=High  T=0 K  T_nominal_specify=off  T_nominal_value=1  T_nominal_unit=K  Q_specify=off  Q_priority=High  Q=0 J/s  Q_nominal_specify=off  Q_nominal_value=1  Q_nominal_unit=W
  Half Wall-Air Conduction : fl_lib/Thermal/Thermal Elements/Conductive Heat Transfer  thermal_type=foundation.enum.ConstantVariableTabulated.Constant  wall_geometry=foundation.enum.ConductionWallGeometry.Planar  area=22 m^2  thickness=.16 m  d_in=0.05 m  d_out=0.1 m  L=1 m  th_cond_min=10 W/(K*m)  th_cond=.069 W/m/K  th_cond_TLU=[413, 401, 392, 383, 371, 357, 342] W/(K*m)  temp_TLU=[200, 273, 400, 600, 800, 1000, 1200] K  T_specify=off  T_priority=High  T=0 K  T_nominal_specify=off  T_nominal_value=1  T_nominal_unit=K  Q_specify=off  Q_priority=High  Q=0 J/s  Q_nominal_specify=off  Q_nominal_value=1  Q_nominal_unit=W
  Half Wall-Atm Conduction : fl_lib/Thermal/Thermal Elements/Conductive Heat Transfer  thermal_type=foundation.enum.ConstantVariableTabulated.Constant  wall_geometry=foundation.enum.ConductionWallGeometry.Planar  area=22 m^2  thickness=.16 m  d_in=0.05 m  d_out=0.1 m  L=1 m  th_cond_min=10 W/(K*m)  th_cond=.069 W/m/K  th_cond_TLU=[413, 401, 392, 383, 371, 357, 342] W/(K*m)  temp_TLU=[200, 273, 400, 600, 800, 1000, 1200] K  T_specify=off  T_priority=High  T=0 K  T_nominal_specify=off  T_nominal_value=1  T_nominal_unit=K  Q_specify=off  Q_priority=High  Q=0 J/s  Q_nominal_specify=off  Q_nominal_value=1  Q_nominal_unit=W
  Half Window-Air Conduction : fl_lib/Thermal/Thermal Elements/Conductive Heat Transfer  thermal_type=foundation.enum.ConstantVariableTabulated.Constant  wall_geometry=foundation.enum.ConductionWallGeometry.Planar  area=5 m^2  thickness=.027 m  d_in=0.05 m  d_out=0.1 m  L=1 m  th_cond_min=10 W/(K*m)  th_cond=.43 W/m/K  th_cond_TLU=[413, 401, 392, 383, 371, 357, 342] W/(K*m)  temp_TLU=[200, 273, 400, 600, 800, 1000, 1200] K  T_specify=off  T_priority=High  T=0 K  T_nominal_specify=off  T_nominal_value=1  T_nominal_unit=K  Q_specify=off  Q_priority=High  Q=0 J/s  Q_nominal_specify=off  Q_nominal_value=1  Q_nominal_unit=W
  Half Window-Atm Conduction : fl_lib/Thermal/Thermal Elements/Conductive Heat Transfer  thermal_type=foundation.enum.ConstantVariableTabulated.Constant  wall_geometry=foundation.enum.ConductionWallGeometry.Planar  area=5 m^2  thickness=.027 m  d_in=0.05 m  d_out=0.1 m  L=1 m  th_cond_min=10 W/(K*m)  th_cond=.43 W/m/K  th_cond_TLU=[413, 401, 392, 383, 371, 357, 342] W/(K*m)  temp_TLU=[200, 273, 400, 600, 800, 1000, 1200] K  T_specify=off  T_priority=High  T=0 K  T_nominal_specify=off  T_nominal_value=1  T_nominal_unit=K  Q_specify=off  Q_priority=High  Q=0 J/s  Q_nominal_specify=off  Q_nominal_value=1  Q_nominal_unit=W
  Thermal Mass Wall : fl_lib/Thermal/Thermal Elements/Thermal Mass  mass_type=foundation.enum.constant_variable.constant  mass=2206 kg  sp_heat=876 J/kg/K  mass_min=1e-6 kg  num_ports=foundation.enum.numPorts2.one  m_specify=off  m_priority=High  m=1 kg  m_nominal_specify=off  m_nominal_value=1  m_nominal_unit=kg  T_specify=on  T_priority=High  T=Ti degC  T_nominal_specify=off  T_nominal_value=1  T_nominal_unit=K  Q_specify=off  Q_priority=None  Q=0 W  Q_nominal_specify=off  Q_nominal_value=1  Q_nominal_unit=W
  Thermal Mass Window : fl_lib/Thermal/Thermal Elements/Thermal Mass  mass_type=foundation.enum.constant_variable.constant  mass=300 kg  sp_heat=884 J/kg/K  mass_min=1e-6 kg  num_ports=foundation.enum.numPorts2.one  m_specify=off  m_priority=High  m=1 kg  m_nominal_specify=off  m_nominal_value=1  m_nominal_unit=kg  T_specify=on  T_priority=High  T=Ti degC  T_nominal_specify=off  T_nominal_value=1  T_nominal_unit=K  Q_specify=off  Q_priority=None  Q=0 W  Q_nominal_specify=off  Q_nominal_value=1  Q_nominal_unit=W
  Conn1 : PMIOPort  Side=Left
  Conn2 : PMIOPort  Port=2  Side=Right
  connections:
  Half Wall-Atm Conduction/RConn1 -- Atm-Wall Convection/LConn1
  Half Window-Atm Conduction/RConn1 -- Atm-Window Convection/LConn1
  Air-Window Convection/RConn1 -- Half Window-Air Conduction/LConn1
  Air-Wall Convection/RConn1 -- Half Wall-Air Conduction/LConn1
  Half Window-Atm Conduction/LConn1 -- Half Window-Air Conduction/RConn1 -- Thermal Mass Window/LConn1
  Half Wall-Atm Conduction/LConn1 -- Half Wall-Air Conduction/RConn1 -- Thermal Mass Wall/LConn1
  Conn1/RConn1 -- Air-Wall Convection/LConn1 -- Air-Window Convection/LConn1
  Atm-Window Convection/RConn1 -- Atm-Wall Convection/RConn1 -- Conn2/RConn1

== system Main_SpeedOptimisedVersionTannenweg/OG2/Raum1/Temp. Sensor ==
  PS2S : nesl_utility/PS-Simulink Converter  PhysicalDomain=network_engine_domain  SubClassName=ps_output  LeftPortType=input  RightPortType=output  PseudoPeriodic=off  Frequencies=[]  VectorFormat=1-D array  Unit=degC  AffineConversion=on
  TRef : fl_lib/Thermal/Thermal Elements/Thermal Reference
  Temperature Sensor : fl_lib/Thermal/Thermal Sensors/Temperature Sensor  temperature_measure=foundation.enum.MeasurementReference.difference
  Pr : PMIOPort  Side=Left
  T : Outport  VectorParamsAs1DForOutWhenUnconnected=off
  wires:
  PS2S/1 -> T/1
  connections:
  Temperature Sensor/RConn1 -- TRef/LConn1
  PS2S/LConn1 -- Temperature Sensor/RConn2
  Pr/RConn1 -- Temperature Sensor/LConn1
